simulink model "Lab4_Task_2"  (R2025b)
settings: Solver=FixedStepAuto  StartTime=0.0  StopTime=inf  RelTol=1e-3
model workspace (MAT data in the model file):
  SL_ROS_VariableLengthArrays_MaxSizes.CommonInfo.ArrayTruncateAction = 'EmitWarning'
  SL_ROS_VariableLengthArrays_MaxSizes.MsgTypeMap = containers.Map
  SL_ROS_VariableLengthArrays_MaxSizes.MsgTypeMap.serialization.keys = {'sensor_msgs/LaserScan'}
  SL_ROS_VariableLengthArrays_MaxSizes.MsgTypeMap.serialization.values{1}(1).PropertyName = 'intensities'
  SL_ROS_VariableLengthArrays_MaxSizes.MsgTypeMap.serialization.values{1}(1).DataType = 'single'
  SL_ROS_VariableLengthArrays_MaxSizes.MsgTypeMap.serialization.values{1}(1).MaxLength = 360
  SL_ROS_VariableLengthArrays_MaxSizes.MsgTypeMap.serialization.values{1}(2).PropertyName = 'ranges'
  SL_ROS_VariableLengthArrays_MaxSizes.MsgTypeMap.serialization.values{1}(2).DataType = 'single'
  SL_ROS_VariableLengthArrays_MaxSizes.MsgTypeMap.serialization.values{1}(2).MaxLength = 360
  SL_ROS_VariableLengthArrays_MaxSizes.MsgTypeMap.serialization.uniformity = 0
  SL_ROS_VariableLengthArrays_MaxSizes.MsgTypeMap.serialization.keyType = 'char'
  SL_ROS_VariableLengthArrays_MaxSizes.MsgTypeMap.serialization.valueType = 'any'
undefined symbols (not defined in the file or in its folder): header, twist
libraries: ros2lib x4
settings Model: Creator=scott  LastModifiedBy=abodynasser22
settings OptimizationCC: DefaultParameterBehavior=Inlined  EnhancedBackFolding=on  PassReuseOutputArgsAs=Individual arguments  ZeroExternalMemoryAtStartup=off  ZeroInternalMemoryAtStartup=off  MaxStackSize=64  OptimizeBlockOrder=speed  DifferentSizesBufferReuse=on  OptimizationCustomize=off  EfficientTunableParamExpr=on
settings DebuggingCC: ParameterTunabilityLossMsg=error
settings HardwareCC: ProdBitPerPointer=32.0  ProdBitPerSizeT=32.0  ProdBitPerPtrDiffT=32.0  ProdWordSize=32.0  ProdHWDeviceType=Intel->x86-32 (Windows32)  UseEmbeddedCoderFeatures=off
settings RTWCC: SystemTargetFile=ert.tlc  HardwareBoard=Robot Operating System 2 (ROS 2)  TLCOptions="-aInlineSetEventsForThisBaseRateFcn=TLC_FALSE -aSuppressMultiTaskScheduler=TLC_FALSE  -aRateBasedStepFcn=0"  TemplateMakefile=ert_default_tmf  Toolchain=Colcon Tools  TargetLang=C++  Description=Embedded Coder
settings CodeAppCC: ForceParamTrailComments=on  IgnoreCustomStorageClasses=off  OperatorAnnotations=on  SimulinkDataObjDesc=on  SFDataObjDesc=on  InsertBlockDesc=on
settings ERTTargetCC: ExtModeTransport=2.0  ExtModeStaticAlloc=on  ExtModeAutomaticAllocSize=off  ExtModeMexFile=ext_xcp  ExtModeIntrfLevel=Level2 - Open  RootIOFormat=Structure reference  CodeInterfacePackaging=C++ class  SupportNonInlinedSFcns=on

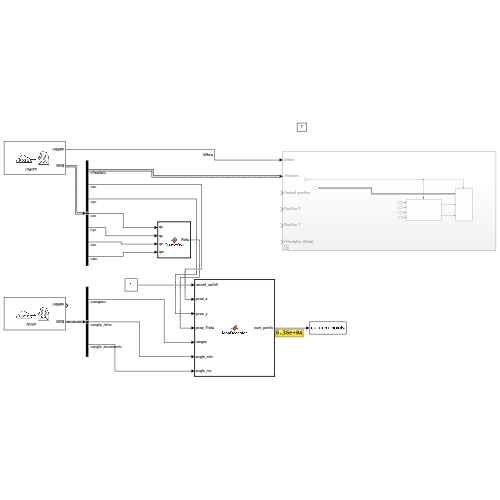
[thumbnail: Simulink's stored preview of the top-level diagram]
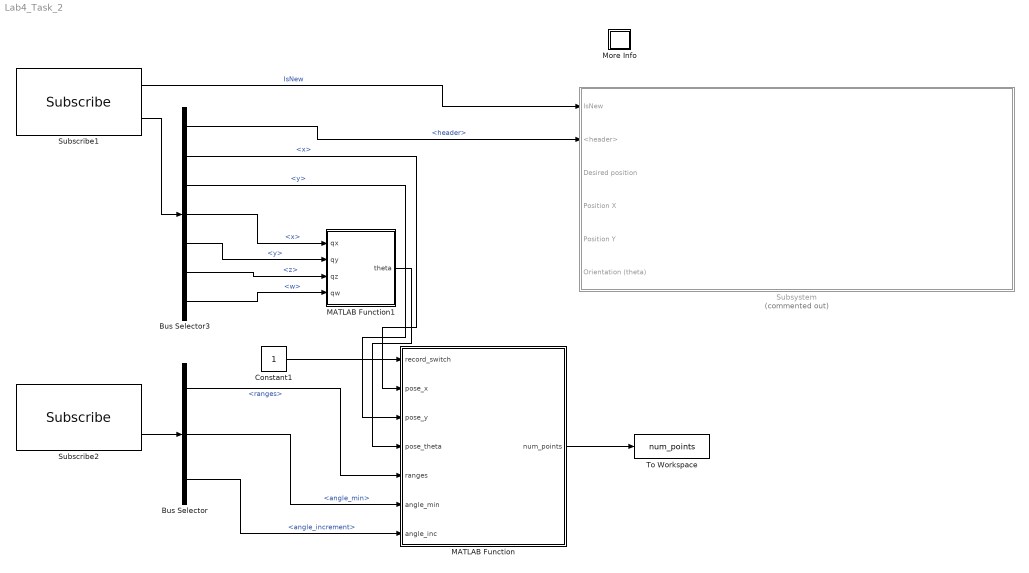
== system Lab4_Task_2 ==
  Bus Selector : BusSelector  OutputSignals=ranges,angle_min,angle_increment
  Bus Selector3 : BusSelector  OutputSignals=header,pose.pose.position.x,pose.pose.position.y,pose.pose.orientation.x,pose.pose.orientation.y,pose.pose.orientation.z,pose.pose.orientation.w
  Constant1 : Constant
  MATLAB Function : MATLAB Function  TreatAsAtomicUnit=on
  MATLAB Function1 : MATLAB Function  TreatAsAtomicUnit=on
  More Info : Subsystem
      settings: OpenFcn=showdemo(bdroot(gcb))
      mask Display: disp('?')
  Subscribe1 : ros2lib/Subscribe  topicSource=Select from ROS network  topic=/odom  messageType=nav_msgs/Odometry  sampleTime=-1  QOSHistory=Keep last  QOSDepth=10  QOSReliability=Reliable  QOSDurability=Volatile  QOSDeadline=Inf  QOSLifespan=Inf  QOSLiveliness=Automatic  QOSLeaseDuration=Inf  QOSAvoidROSNamespaceConventions=off
  Subscribe2 : ros2lib/Subscribe  topicSource=Select from ROS network  topic=/scan  messageType=sensor_msgs/LaserScan  sampleTime=-1  QOSHistory=Keep last  QOSDepth=10  QOSReliability=Best effort  QOSDurability=Volatile  QOSDeadline=Inf  QOSLifespan=Inf  QOSLiveliness=Automatic  QOSLeaseDuration=Inf  QOSAvoidROSNamespaceConventions=off
  Subsystem : Subsystem  Commented=on
  To Workspace : ToWorkspace  VariableName=num_points  SaveFormat=Timeseries  SampleTime=-1
  wires:
  Subscribe1/2 -> Bus Selector3/1
  Bus Selector3/2 -> MATLAB Function/2(pose_x)  "<x>"
  Bus Selector3/3 -> MATLAB Function/3(pose_y)  "<y>"
  Bus Selector3/4 -> MATLAB Function1/1(qx)  "<x>"
  Bus Selector3/5 -> MATLAB Function1/2(qy)  "<y>"
  Bus Selector3/6 -> MATLAB Function1/3(qz)  "<z>"
  Bus Selector3/7 -> MATLAB Function1/4(qw)  "<w>"
  Subscribe2/2 -> Bus Selector/1
  Bus Selector/1 -> MATLAB Function/5(ranges)  "<ranges>"
  Bus Selector/2 -> MATLAB Function/6(angle_min)  "<angle_min>"
  Bus Selector/3 -> MATLAB Function/7(angle_inc)  "<angle_increment>"
  MATLAB Function1/1(theta) -> MATLAB Function/4(pose_theta)
  Constant1/1 -> MATLAB Function/1(record_switch)
  MATLAB Function/1(num_points) -> To Workspace/1
  Subscribe1/1 -> Subsystem/1(IsNew)  "IsNew"
  Bus Selector3/1 -> Subsystem/2(<header>)  "<header>"

== system Lab4_Task_2/More Info ==

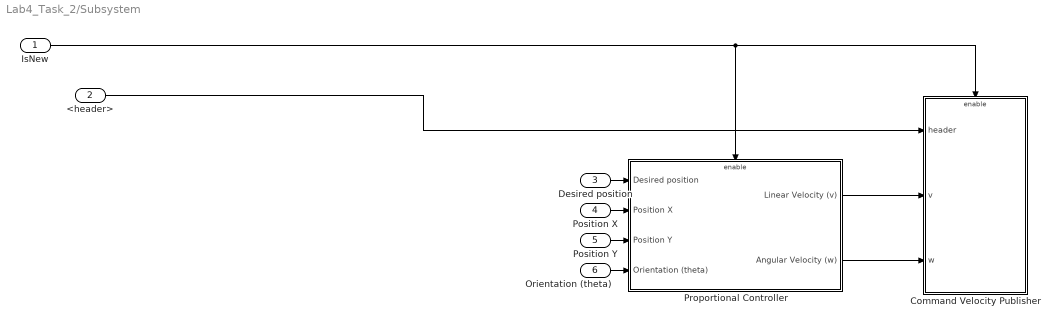
== system Lab4_Task_2/Subsystem ==
  IsNew : Inport
  <header> : Inport  Port=2
  Desired position : Inport  Port=3
  Position X : Inport  Port=4
  Position Y : Inport  Port=5
  Orientation (theta) : Inport  Port=6
  Command Velocity Publisher : Subsystem
  Proportional Controller : Subsystem
  wires:
  Orientation (theta)/1 -> Proportional Controller/4(Orientation (theta))
  Position Y/1 -> Proportional Controller/3(Position Y)
  <header>/1 -> Command Velocity Publisher/1(header)
  Position X/1 -> Proportional Controller/2(Position X)
  Proportional Controller/1(Linear Velocity (v)) -> Command Velocity Publisher/2(v)
  Proportional Controller/2(Angular Velocity (w)) -> Command Velocity Publisher/3(w)
  Desired position/1 -> Proportional Controller/1(Desired position)
  IsNew/1 -> Command Velocity Publisher/Enable, Proportional Controller/Enable

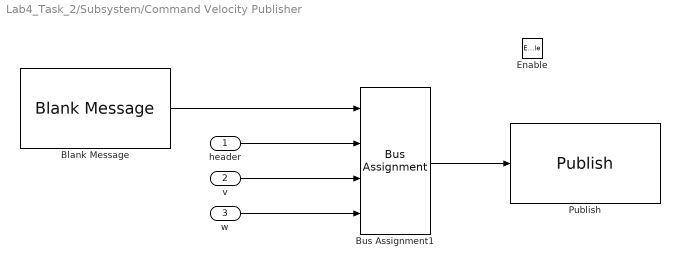
== system Lab4_Task_2/Subsystem/Command Velocity Publisher ==
  header : Inport
  v : Inport  Port=2
  w : Inport  Port=3
  Enable : EnablePort
  Blank Message : ros2lib/Blank Message  messageClass=Message  entityType=geometry_msgs/TwistStamped  messageType=geometry_msgs/TwistStamped  SampleTime=inf
  Bus Assignment1 : BusAssignment  DialogController=Simulink.DDGSource_BusAssignment  AssignedSignals=header,twist.linear.x,twist.angular.z
  Publish : ros2lib/Publish  topicSource=Select from ROS network  topic=/cmd_vel  messageType=geometry_msgs/TwistStamped  QOSHistory=Keep last  QOSDepth=10  QOSReliability=Reliable  QOSDurability=Volatile  QOSDeadline=Inf  QOSLifespan=Inf  QOSLiveliness=Automatic  QOSLeaseDuration=Inf  QOSAvoidROSNamespaceConventions=off
  wires:
  Bus Assignment1/1 -> Publish/1
  Blank Message/1 -> Bus Assignment1/1
  header/1 -> Bus Assignment1/2
  v/1 -> Bus Assignment1/3
  w/1 -> Bus Assignment1/4

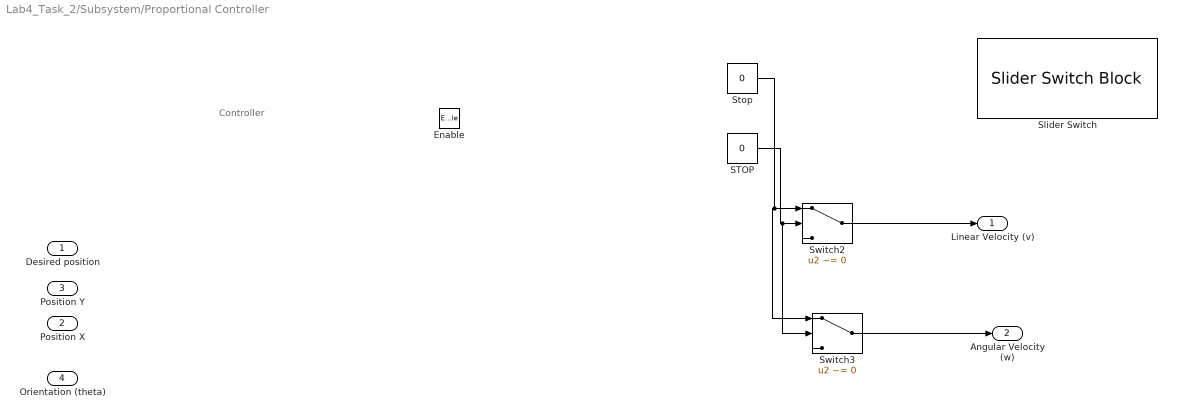
== system Lab4_Task_2/Subsystem/Proportional Controller ==
  note: Controller
  Desired position : Inport
  Position X : Inport  Port=2
  Position Y : Inport  Port=3
  Orientation (theta) : Inport  Port=4
  Enable : EnablePort
  "STOP " : Constant  Value=0
  Slider Switch : SliderSwitchBlock
  Stop : Constant  Value=0
  Switch2 : Switch  Criteria=u2 ~= 0  SaturateOnIntegerOverflow=off  InputSameDT=off
  Switch3 : Switch  Criteria=u2 ~= 0  SaturateOnIntegerOverflow=off  InputSameDT=off
  Linear Velocity (v) : Outport  VectorParamsAs1DForOutWhenUnconnected=off
  Angular Velocity (w) : Outport  Port=2  VectorParamsAs1DForOutWhenUnconnected=off
  wires:
  Stop/1 -> Switch3/1, Switch2/1
  "STOP "/1 -> Switch3/2, Switch2/2
  Switch2/1 -> Linear Velocity (v)/1
  Switch3/1 -> Angular Velocity (w)/1

== matlab function Lab4_Task_2/MATLAB Function1 ==
  data: qx input; theta output; qy input; qz input; qw input
function theta = Quat2Yaw(qx, qy, qz, qw)
%#codegen
% Inputs are quaternion components from /odom:
% orientation.x = qx, .y = qy, .z = qz, .w = qw

% Build 1x4 quaternion row in the order [w x y z]
q = [qw, qx, qy, qz];

% Convert to Euler angles [yaw pitch roll] (ZYX convention)
eul = quat2eul(q, 'ZYX');

% Use yaw (rotation about Z-axis)
theta = eul(1);
end

== matlab function Lab4_Task_2/MATLAB Function ==
  data: record_switch input; pose_x input; pose_y input; pose_theta input; ranges input; num_points output; angle_min input; angle_inc input
function num_points = MapRecorder(record_switch, pose_x, pose_y, pose_theta, ranges, angle_min, angle_inc)
    %#codegen
    persistent map_points last_save_time
    
    if isempty(map_points)
        map_points = zeros(0, 2);
    end
    if isempty(last_save_time)
        last_save_time = 0;
    end
    
    % Only record if the switch is ON (1)
    if record_switch == 1
        ranges = double(ranges);
        
        % DOWNSAMPLING: Only take every 3rd ray to save memory
        % The Lidar is high-res enough that we don't need all 360 points
        indices = 1:3:numel(ranges); 
        
        r_sub = ranges(indices);
        
        % Filter Data
        valid_mask = (r_sub > 0.1) & (r_sub < 3.5) & ~isinf(r_sub);
        
        if any(valid_mask)
            r_valid = r_sub(valid_mask);
            
            % Calculate Angles (Vectorized)
            % Note: Check your indices alignment carefully
            idx_valid = indices(valid_mask) - 1; 
            angles_local = double(angle_min) + idx_valid' * double(angle_inc);
            angles_global = angles_local + pose_theta;
            
            % Polar to Cartesian
            x_obs = pose_x + r_valid .* cos(angles_global);
            y_obs = pose_y + r_valid .* sin(angles_global);
            
            % Append
            new_points = [x_obs, y_obs];
            map_points = [map_points; new_points];
        end
        
        % SAVE LOGIC: Only export to workspace every 50 iterations (approx 0.5 sec)
        % This prevents the simulation from lagging due to "assignin" overhead
        last_save_time = last_save_time + 1;
        if last_save_time > 50
            assignin('base', 'collected_map_points', map_points);
            last_save_time = 0;
        end
    end
    
    num_points = size(map_points, 1);
end
